simulink model "rlwatertankPIDTune"  (R2025b)
settings: Solver=ode45  StartTime=0.0  StopTime=200  RelTol=1e-3  EnableMultiTasking=on
undefined symbols (not defined in the file): DiscIntNeverNeededParam, Href, Ts
libraries: rllib x1
settings Model: Creator=The MathWorks, Inc.  LastModifiedBy=The MathWorks, Inc.
settings SolverCC: AlgebraicLoopSolver=TrustRegion  MaxZcPerStep=1.0
settings DataIOCC: LimitDataPoints=on  SaveFormat=Array  SignalLoggingName=logsOut
settings OptimizationCC: ExpressionDepthLimit=2147483647.0  InitFltsAndDblsToZero=on  LifeSpan=inf
settings DebuggingCC: SaveWithParameterizedLinksMsg=none  UnderspecifiedInitializationDetection=Classic  MergeDetectMultiDrivingBlocksExec=none  SignalResolutionControl=TryResolveAllWithWarning  MultiTaskDSMMsg=warning  FcnCallInpInsideContextMsg=warning  UnconnectedInputMsg=warning  UnconnectedOutputMsg=warning  UnconnectedLineMsg=warning  AllowSymbolicDim=off  StateNameClashWarn=warning  SFUnexpectedBacktrackingDiag=warning  SFNoUnconditionalDefaultTransitionDiag=warning  SFExecutionAtInitializationDiag=none  ArithmeticOperatorsInVariantConditions=warning
settings HardwareCC: ProdBitPerPointer=32.0  ProdBitPerSizeT=32.0  ProdBitPerPtrDiffT=32.0  ProdLargestAtomicFloat=None  ProdIntDivRoundTo=Undefined  ProdEndianess=Unspecified  ProdWordSize=32.0  ProdHWDeviceType=Specified
settings ModelReferenceCC: EnableRefExpFcnMdlSchedulingChecks=on  PropagateSignalLabelsOutOfModel=off
settings SFSimCC: SimUseLocalCustomCode=off
settings RTWCC: RTWUseLocalCustomCode=off  GPUComputeCapability=3.5  DLArmComputeVersion=19.05
settings CodeAppCC: StateflowObjectComments=on
settings GRTTargetCC: TargetFcnLib=ansi_tfl_tmw.mat  TargetLangStandard=C89/C90 (ANSI)  CombineOutputUpdateFcns=off  GRTInterface=on
settings ConfigComp: CovMetricSettings=dw  CovSaveCumulativeToWorkspaceVar=on  CovSaveSingleToWorkspaceVar=on  CovExternalEMLEnable=off

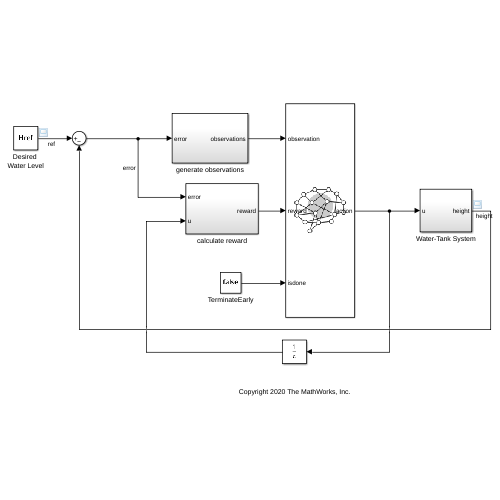
[thumbnail: Simulink's stored preview of the top-level diagram]
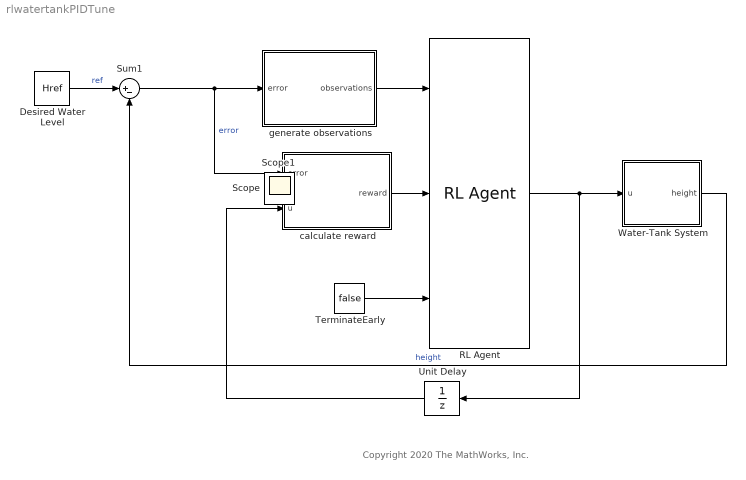
== system rlwatertankPIDTune ==
  note: Copyright 2020 The MathWorks, Inc.
  Desired Water Level : Constant  Value=Href
  RL Agent : rllib/RL Agent  Agent=agent  ExternalActionAsInput=off  ProvideLastAction=off  ProvideCumRwd=off  TreatAsDirectFeedthrough=on  UseStrictObservationDataTypes=off
  Sum1 : Sum  Inputs=|+-  SaturateOnIntegerOverflow=on
  TerminateEarly : Constant  Value=false
  Unit Delay : UnitDelay  SampleTime=-1  HasFrameUpgradeWarning=on
  Water-Tank System : Subsystem
  calculate reward : Subsystem
  generate observations : Subsystem
  Scope : Scope
      settings: ActiveDisplayYMinimum=0.26116  ActiveDisplayYMaximum=2.71198
  Scope1 : Scope
  wires:
  Desired Water Level/1 -> Sum1/1  "ref"
  Sum1/1 -> calculate reward/1(error), generate observations/1(error)  "error"
  generate observations/1(observations) -> RL Agent/1
  RL Agent/1 -> Unit Delay/1, Water-Tank System/1(u)
  Water-Tank System/1(height) -> Sum1/2  "height"
  Unit Delay/1 -> calculate reward/2(u)
  calculate reward/1(reward) -> RL Agent/2
  TerminateEarly/1 -> RL Agent/3

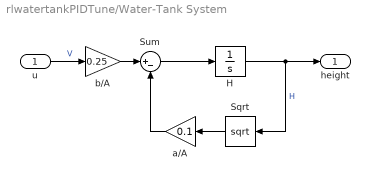
== system rlwatertankPIDTune/Water-Tank System ==
  u : Inport
  H : Integrator  InitialCondition=10.2886  LimitOutput=on  LowerSaturationLimit=0
  Sqrt : Sqrt  OutputSignalType=real
  Sum : Sum  Inputs=|+-  SaturateOnIntegerOverflow=on
  a/A : Gain  Gain=0.1  SaturateOnIntegerOverflow=on  OutDataTypeStr=Inherit: Same as input  ParamDataTypeStr=Inherit: Same as input
  b/A : Gain  Gain=0.25  SaturateOnIntegerOverflow=on  OutDataTypeStr=Inherit: Same as input  ParamDataTypeStr=Inherit: Same as input
  height : Outport  VectorParamsAs1DForOutWhenUnconnected=off
  wires:
  b/A/1 -> Sum/1
  Sum/1 -> H/1
  H/1 -> Sqrt/1, height/1  "H"
  Sqrt/1 -> a/A/1
  a/A/1 -> Sum/2
  u/1 -> b/A/1  "V"

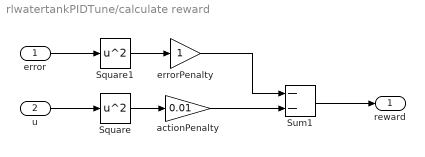
== system rlwatertankPIDTune/calculate reward ==
  error : Inport
  u : Inport  Port=2
  Square : Math  Operator=square
  Square1 : Math  Operator=square
  Sum1 : Sum  Inputs=--  OutDataTypeStr=double
  actionPenalty : Gain  Gain=0.01
  errorPenalty : Gain
  reward : Outport  VectorParamsAs1DForOutWhenUnconnected=off
  wires:
  Square1/1 -> errorPenalty/1
  errorPenalty/1 -> Sum1/1
  actionPenalty/1 -> Sum1/2
  Square/1 -> actionPenalty/1
  u/1 -> Square/1
  error/1 -> Square1/1
  Sum1/1 -> reward/1

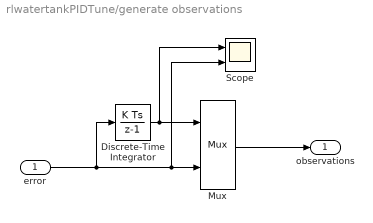
== system rlwatertankPIDTune/generate observations ==
  error : Inport
  Discrete-Time Integrator : DiscreteIntegrator  SampleTime=Ts  ICPrevOutput=DiscIntNeverNeededParam  ICPrevScaledInput=DiscIntNeverNeededParam
  Mux : Mux  Inputs=2
  Scope : Scope  NumInputPorts=2
      settings: ActiveDisplayYMinimum=-2.63404  ActiveDisplayYMaximum=11.10792  DataLoggingVariableName=ScopeData2
  observations : Outport  VectorParamsAs1DForOutWhenUnconnected=off
  wires:
  Discrete-Time Integrator/1 -> Scope/1, Mux/1
  error/1 -> Discrete-Time Integrator/1, Scope/2, Mux/2
  Mux/1 -> observations/1
